simulink model "Simulink_Motor_model_working"  (R2026a)
settings: Solver=VariableStepAuto  MaxStep=0.001
values from neighbouring files (symbols this model uses):
  B = 0.15    [Motor_model_param.m]
  D = 3.323e-6    (= 3.323e-06)    [Motor_model_param.m]
  gear = 9.68    [Motor_model_param.m]
  head_alpha = 0.5    [Motor_model_param.m]
  head_tau_d = 0.8    [Motor_model_param.m]
  J = 5.4619e-6    (= 5.4619e-06)    [Motor_model_param.m]
  Kb = Kt    (= 0.007956)    [Motor_model_param.m]
  Ki_vel_left = 0.1    [Motor_model_param.m]
  Ki_vel_right = 0.1    [Motor_model_param.m]
  Kp_vel_left = 0.05    [Motor_model_param.m]
  Kp_vel_right = 0.04    [Motor_model_param.m]
  Kph = 2.5    [Motor_model_param.m]
  KpLT = 25    [Motor_model_param.m]
  KpLV = 25    [Motor_model_param.m]
  Kt = 0.007956    [Motor_model_param.m]
  L = 0.00380    (= 0.0038)    [Motor_model_param.m]
  Lim_TL = -0.7    [Motor_model_param.m]
  Lim_TU = 0.7    [Motor_model_param.m]
  Lim_VL = -0.5    [Motor_model_param.m]
  Lim_VU = 0.5    [Motor_model_param.m]
  R = 2.84    [Motor_model_param.m]
  uh = 1    [Motor_model_param.m]
  wrad = 0.03    [Motor_model_param.m]
settings Model: Creator=mariu  LastModifiedBy=mariu

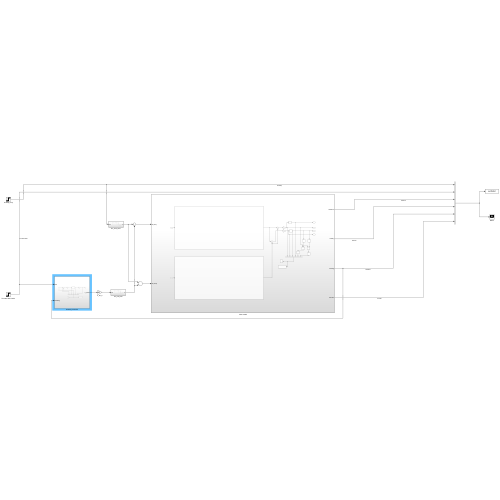
[thumbnail: Simulink's stored preview of the top-level diagram]
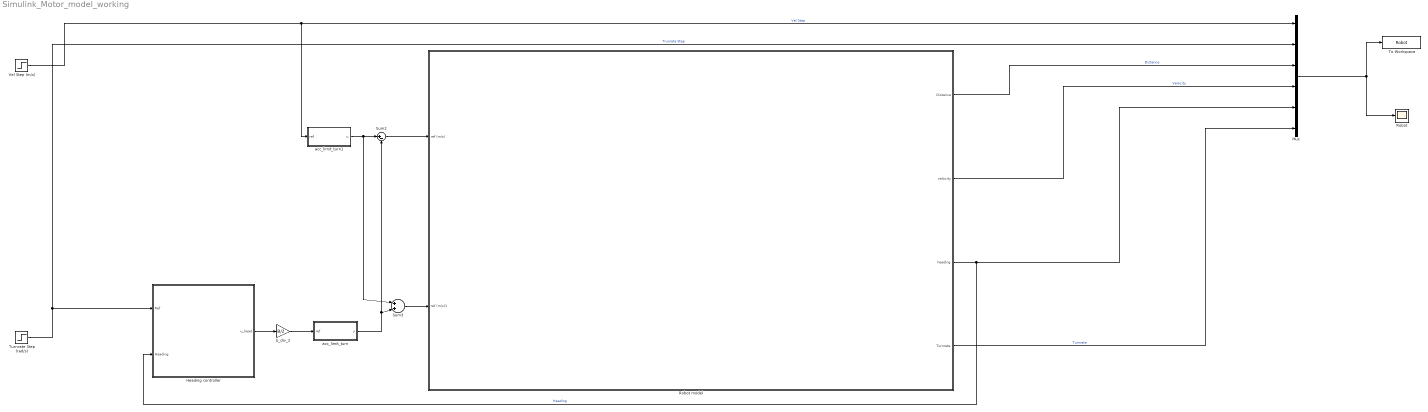
== system Simulink_Motor_model_working ==
  Heading controller : Subsystem
  Mux : Mux  Inputs=6
  Robot : Scope
      settings: ActiveDisplayYMinimum=-5.8842376520189088  ActiveDisplayYMaximum=10.788459335212691
  Robot model : Subsystem
  Sum2 : Sum  Inputs=|+-
  Sum3 : Sum  Inputs=|++|
  To Workspace : ToWorkspace  VariableName=Robot  SaveFormat=Timeseries  SampleTime=-1
  Turnrate Step (rad/s) : Step  Time=0.5  SampleTime=0
  Vel Step (m/s) : Step  Time=0.1  FinalValue=0.6  SampleTime=0
  acc_limit_turn : Subsystem
  acc_limit_turn1 : Subsystem
  b_div_2 : Gain  Gain=B/2
  wires:
  Robot model/1(Distance) -> Mux/3  "Distance"
  Robot model/2(velocity) -> Mux/4  "Velocity"
  Robot model/3(heading) -> Heading controller/2(Heading), Mux/5  "Heading"
  Robot model/4(Turnrate) -> Mux/6  "Turnrate"
  Vel Step (m/s)/1 -> acc_limit_turn1/1(ref), Mux/1  "Vel Step"
  Turnrate Step (rad/s)/1 -> Heading controller/1(Ref), Mux/2  "Trunrate Step"
  Mux/1 -> To Workspace/1, Robot/1
  Sum2/1 -> Robot model/1(ref (m/s))
  Sum3/1 -> Robot model/2(ref (m/s)1)
  acc_limit_turn/1(u) -> Sum2/2, Sum3/2
  acc_limit_turn1/1(u) -> Sum3/1, Sum2/1
  Heading controller/1(u_head) -> b_div_2/1
  b_div_2/1 -> acc_limit_turn/1(ref)

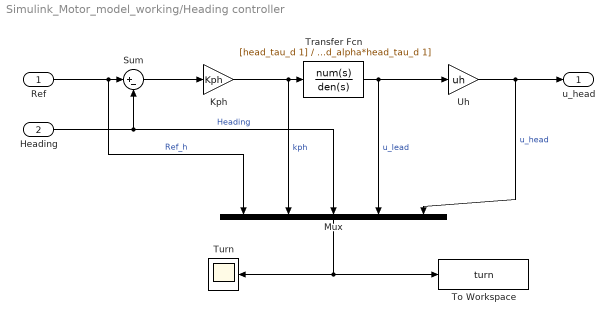
== system Simulink_Motor_model_working/Heading controller ==
  Ref : Inport
  Heading : Inport  Port=2
  Kph : Gain  Gain=Kph
  Mux : Mux  Inputs=5
  Sum : Sum  Inputs=|+-
  To Workspace : ToWorkspace  VariableName=turn  SaveFormat=Timeseries  SampleTime=-1
  Transfer Fcn : TransferFcn  Numerator=[head_tau_d 1]  Denominator=[head_alpha*head_tau_d 1]
  Turn : Scope
      settings: ActiveDisplayYMinimum=-21.899520221389576  ActiveDisplayYMaximum=44.638128708270415  DataLoggingVariableName=ScopeData2
  Uh : Gain  Gain=uh
  u_head : Outport
  wires:
  Ref/1 -> Mux/1, Sum/1  "Ref_h"
  Sum/1 -> Kph/1
  Kph/1 -> Mux/2, Transfer Fcn/1  "kph"
  Transfer Fcn/1 -> Uh/1, Mux/4  "u_lead"
  Uh/1 -> Mux/5, u_head/1  "u_head"
  Heading/1 -> Mux/3, Sum/2  "Heading"
  Mux/1 -> Turn/1, To Workspace/1

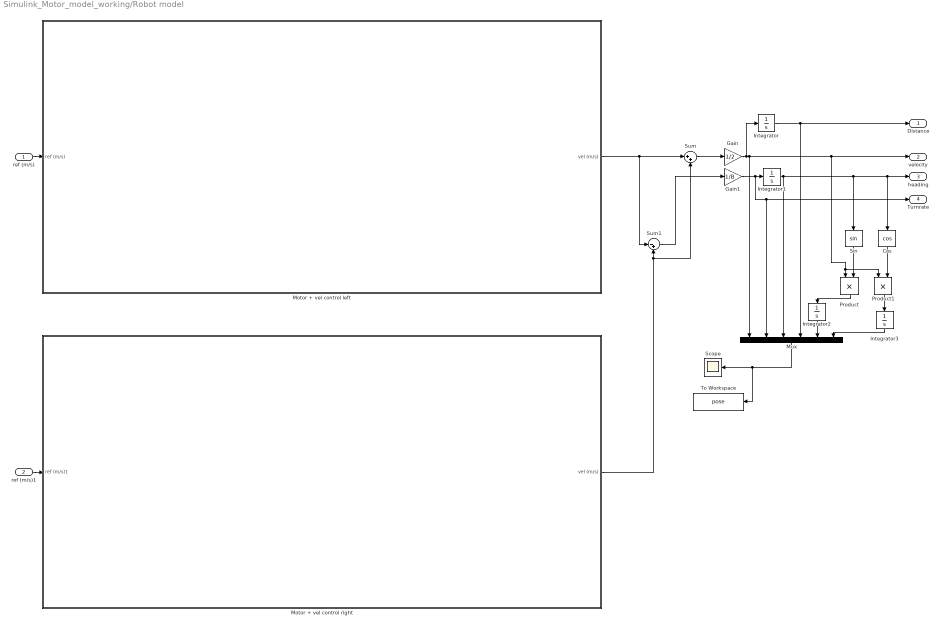
== system Simulink_Motor_model_working/Robot model ==
  ref (m/s) : Inport
  ref (m/s)1 : Inport  Port=2
  Cos : Trigonometry  Operator=cos
  Gain : Gain  Gain=1/2
  Gain1 : Gain  Gain=1/B
  Integrator{,1..3} (4 alike) : Integrator
  Motor + vel control left : Subsystem
  Motor + vel control right : Subsystem
  Mux : Mux  Inputs=6
  Product : Product
  Product1 : Product
  Scope : Scope
      settings: ActiveDisplayYMinimum=-0.1149883215671369  ActiveDisplayYMaximum=0.30477624997481578
  Sin : Trigonometry
  Sum : Sum  Inputs=|++
  Sum1 : Sum  Inputs=|-+
  To Workspace : ToWorkspace  VariableName=pose  SaveFormat=Timeseries  SampleTime=-1
  Distance : Outport
  velocity : Outport  Port=2
  heading : Outport  Port=3
  Turnrate : Outport  Port=4
  wires:
  Integrator1/1 -> Mux/3, Sin/1, heading/1, Cos/1
  Motor + vel control left/1(vel (m/s)) -> Sum1/1, Sum/1
  Gain/1 -> Mux/1, velocity/1, Product1/1, Product/1, Integrator/1
  Gain1/1 -> Turnrate/1, Mux/2, Integrator1/1
  Integrator3/1 -> Mux/6
  Motor + vel control right/1(vel (m/s)) -> Sum/2, Sum1/2
  Product1/1 -> Integrator3/1
  Mux/1 -> To Workspace/1, Scope/1
  Sum/1 -> Gain/1
  Integrator/1 -> Distance/1, Mux/4
  Sin/1 -> Product/2
  Integrator2/1 -> Mux/5
  Sum1/1 -> Gain1/1
  Cos/1 -> Product1/2
  Product/1 -> Integrator2/1
  ref (m/s)1/1 -> Motor + vel control right/1(ref (m/s)1)
  ref (m/s)/1 -> Motor + vel control left/1(ref (m/s))

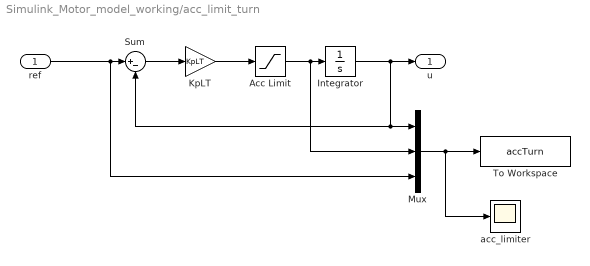
== system Simulink_Motor_model_working/acc_limit_turn ==
  ref : Inport
  Acc Limit : Saturate  UpperLimit=Lim_TU  LowerLimit=Lim_TL
  Integrator : Integrator
  KpLT : Gain  Gain=KpLT
  Mux : Mux  Inputs=3
  Sum : Sum  Inputs=|+-
  To Workspace : ToWorkspace  VariableName=accTurn  SaveFormat=Timeseries  SampleTime=-1
  acc_limiter : Scope
      settings: DataLoggingVariableName=ScopeData3
  u : Outport
  wires:
  ref/1 -> Mux/3, Sum/1
  Sum/1 -> KpLT/1
  KpLT/1 -> Acc Limit/1
  Integrator/1 -> Sum/2, Mux/1, u/1
  Acc Limit/1 -> Mux/2, Integrator/1
  Mux/1 -> To Workspace/1, acc_limiter/1

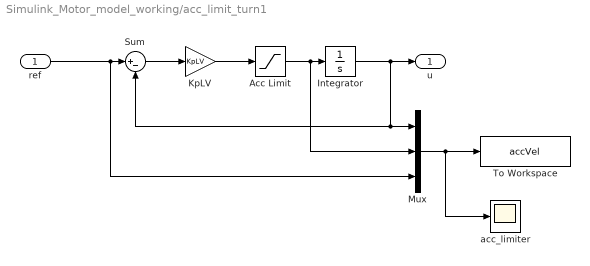
== system Simulink_Motor_model_working/acc_limit_turn1 ==
  ref : Inport
  Acc Limit : Saturate  UpperLimit=Lim_VU  LowerLimit=Lim_VL
  Integrator : Integrator
  KpLV : Gain  Gain=KpLV
  Mux : Mux  Inputs=3
  Sum : Sum  Inputs=|+-
  To Workspace : ToWorkspace  VariableName=accVel  SaveFormat=Timeseries  SampleTime=-1
  acc_limiter : Scope
      settings: DataLoggingVariableName=ScopeData3
  u : Outport
  wires:
  ref/1 -> Mux/3, Sum/1
  Sum/1 -> KpLV/1
  KpLV/1 -> Acc Limit/1
  Integrator/1 -> Sum/2, Mux/1, u/1
  Acc Limit/1 -> Mux/2, Integrator/1
  Mux/1 -> To Workspace/1, acc_limiter/1

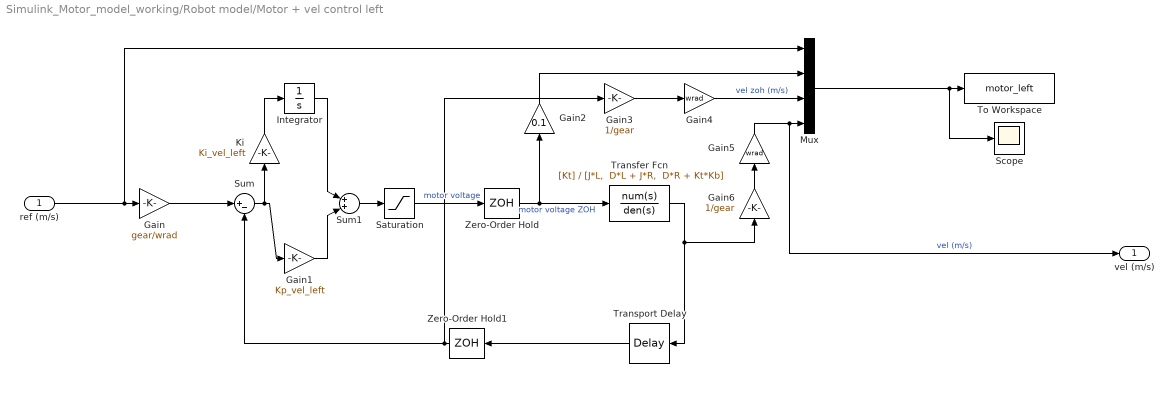
== system Simulink_Motor_model_working/Robot model/Motor + vel control left ==
  ref (m/s) : Inport
  Gain : Gain  Gain=gear/wrad
  Gain1 : Gain  Gain=Kp_vel_left
  Gain2 : Gain  Gain=0.1
  Gain3 : Gain  Gain=1/gear
  Gain4 : Gain  Gain=wrad
  Gain5 : Gain  Gain=wrad
  Gain6 : Gain  Gain=1/gear
  Integrator : Integrator
  Ki : Gain  Gain=Ki_vel_left
  Mux : Mux
  Saturation : Saturate  UpperLimit=9  LowerLimit=-9
  Scope : Scope
      settings: ActiveDisplayYMinimum=-3.3505218283230835  ActiveDisplayYMaximum=3.5845676115773961
  Sum : Sum  Inputs=|+-
  Sum1 : Sum  Inputs=|++|
  To Workspace : ToWorkspace  VariableName=motor_left  SaveFormat=Timeseries  SampleTime=-1
  Transfer Fcn : TransferFcn  Numerator=[Kt]  Denominator="[J*L,  D*L + J*R,  D*R + Kt*Kb]"
  Transport Delay : TransportDelay  DelayTime=0.01
  Zero-Order Hold : ZeroOrderHold  SampleTime=-1
  Zero-Order Hold1 : ZeroOrderHold  SampleTime=-1
  vel (m/s) : Outport
  wires:
  Gain5/1 -> vel (m/s)/1, Mux/4  "vel (m/s)"
  Zero-Order Hold/1 -> Transfer Fcn/1, Gain2/1  "motor voltage ZOH"
  Gain4/1 -> Mux/3  "vel zoh (m/s)"
  Mux/1 -> Scope/1, To Workspace/1
  Gain6/1 -> Gain5/1
  Gain2/1 -> Mux/2
  Transfer Fcn/1 -> Gain6/1, Transport Delay/1
  Gain3/1 -> Gain4/1
  Zero-Order Hold1/1 -> Gain3/1, Sum/2
  ref (m/s)/1 -> Mux/1, Gain/1
  Transport Delay/1 -> Zero-Order Hold1/1
  Saturation/1 -> Zero-Order Hold/1  "motor voltage"
  Gain/1 -> Sum/1
  Sum/1 -> Gain1/1, Ki/1
  Sum1/1 -> Saturation/1
  Gain1/1 -> Sum1/2
  Integrator/1 -> Sum1/1
  Ki/1 -> Integrator/1

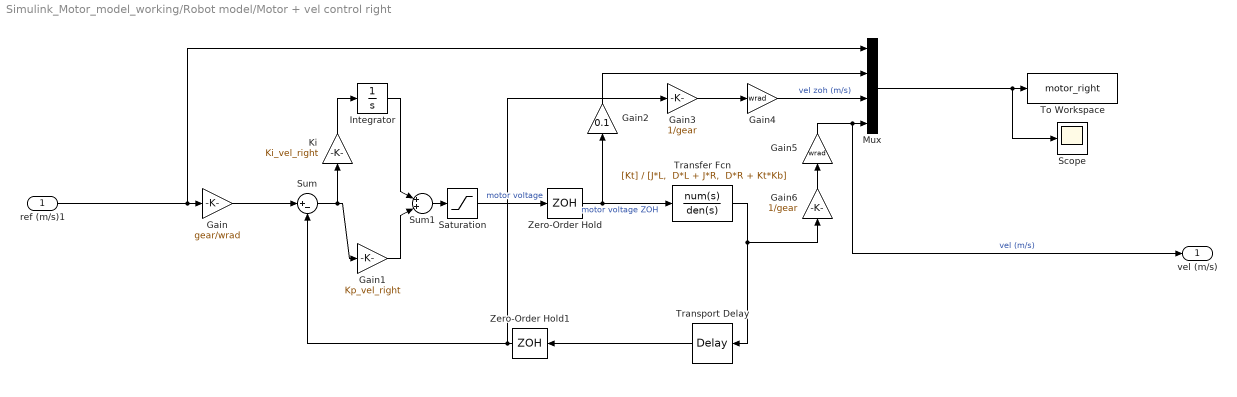
== system Simulink_Motor_model_working/Robot model/Motor + vel control right ==
  ref (m/s)1 : Inport
  Gain : Gain  Gain=gear/wrad
  Gain1 : Gain  Gain=Kp_vel_right
  Gain2 : Gain  Gain=0.1
  Gain3 : Gain  Gain=1/gear
  Gain4 : Gain  Gain=wrad
  Gain5 : Gain  Gain=wrad
  Gain6 : Gain  Gain=1/gear
  Integrator : Integrator
  Ki : Gain  Gain=Ki_vel_right
  Mux : Mux
  Saturation : Saturate  UpperLimit=9  LowerLimit=-9
  Scope : Scope
      settings: ActiveDisplayYMinimum=-1.5972367196499144  ActiveDisplayYMaximum=3.2452747464991383
  Sum : Sum  Inputs=|+-
  Sum1 : Sum  Inputs=|++|
  To Workspace : ToWorkspace  VariableName=motor_right  SaveFormat=Timeseries  SampleTime=-1
  Transfer Fcn : TransferFcn  Numerator=[Kt]  Denominator="[J*L,  D*L + J*R,  D*R + Kt*Kb]"
  Transport Delay : TransportDelay  DelayTime=0.01
  Zero-Order Hold : ZeroOrderHold  SampleTime=-1
  Zero-Order Hold1 : ZeroOrderHold  SampleTime=-1
  vel (m/s) : Outport
  wires:
  Gain5/1 -> vel (m/s)/1, Mux/4  "vel (m/s)"
  Zero-Order Hold/1 -> Transfer Fcn/1, Gain2/1  "motor voltage ZOH"
  Gain4/1 -> Mux/3  "vel zoh (m/s)"
  Mux/1 -> Scope/1, To Workspace/1
  Gain6/1 -> Gain5/1
  Gain2/1 -> Mux/2
  Transfer Fcn/1 -> Gain6/1, Transport Delay/1
  Gain3/1 -> Gain4/1
  Zero-Order Hold1/1 -> Gain3/1, Sum/2
  ref (m/s)1/1 -> Mux/1, Gain/1
  Transport Delay/1 -> Zero-Order Hold1/1
  Saturation/1 -> Zero-Order Hold/1  "motor voltage"
  Gain/1 -> Sum/1
  Integrator/1 -> Sum1/1
  Sum/1 -> Gain1/1, Ki/1
  Gain1/1 -> Sum1/2
  Ki/1 -> Integrator/1
  Sum1/1 -> Saturation/1
